simulink model "mod_fm"  (R2024b)
settings: Solver=FixedStepDiscrete  StartTime=0.0  StopTime=0.05  FixedStep=5e-06  RelTol=1e-3
model workspace (MAT data in the model file):
  df = 5000
  fc = 10000
  fm = 1000
  fs = 200000
  hpost = [-1.25061059478e-19 -3.24125186585e-05 -6.55214055151e-05 -9.93614444025e-05 -0.000133925361151 -0.000169142005337 -0.000204855936976 -0.00024080932373 -0.0002766270145 -0.000311805588382 -0.000345707084751 -0.000377558002721 ... (201 elements, 1x201)]
  hpre = [-2.4993987069e-19 -6.42670110592e-05 -0.000126833377255 -0.000184633240487 -0.000234548351952 -0.000273478101959 -0.00029844948245 -0.000306771591638 -0.000296232329902 -0.000265327256793 -0.000213503048842 -0.000141391531522 ... (201 elements, 1x201)]
  phi = 0.7
  sigma2 = 0.02
undefined symbols (not defined in the file): DiscIntNeverNeededParam
settings Model: Creator=runner  LastModifiedBy=runner

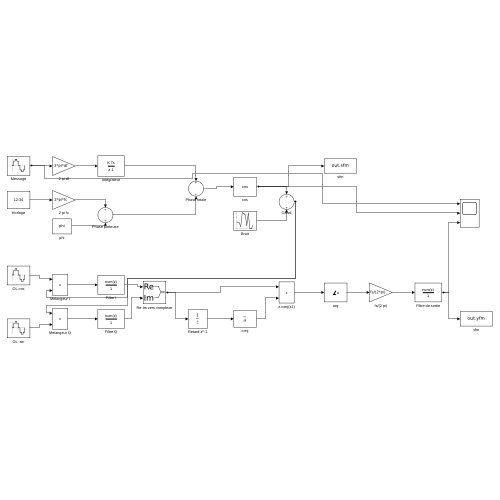
[thumbnail: Simulink's stored preview of the top-level diagram]
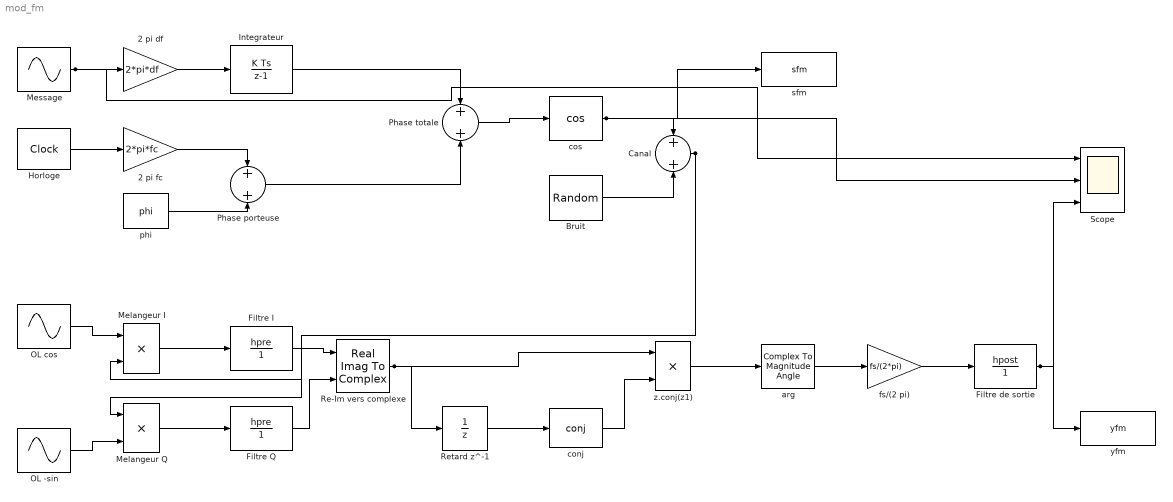
== system mod_fm ==
  2 pi df : Gain  Gain=2*pi*df
  2 pi fc : Gain  Gain=2*pi*fc
  Bruit : RandomNumber  Variance=sigma2  Seed=1  SampleTime=1/fs
  Canal : Sum
  Filtre I : DiscreteFilter  Numerator=hpre  Denominator=1
  Filtre Q : DiscreteFilter  Numerator=hpre  Denominator=1
  Filtre de sortie : DiscreteFilter  Numerator=hpost  Denominator=1
  Horloge : DigitalClock  SampleTime=1/fs
  Integrateur : DiscreteIntegrator  gainval=1  SampleTime=1/fs  ICPrevOutput=DiscIntNeverNeededParam  ICPrevScaledInput=DiscIntNeverNeededParam
  Melangeur I : Product
  Melangeur Q : Product
  Message : Sin  Frequency=2*pi*fm  Phase=pi/2  SampleTime=1/fs
  OL -sin : Sin  Amplitude=-2  Frequency=2*pi*fc  SampleTime=1/fs
  OL cos : Sin  Amplitude=2  Frequency=2*pi*fc  Phase=pi/2  SampleTime=1/fs
  Phase porteuse : Sum
  Phase totale : Sum
  Re-Im vers complexe : RealImagToComplex
  Retard z^-1 : UnitDelay  SampleTime=-1  HasFrameUpgradeWarning=on
  Scope : Scope  NumInputPorts=3
  arg : ComplexToMagnitudeAngle  Output=Angle
  conj : Math  Operator=conj
  cos : Trigonometry  Operator=cos
  fs/(2 pi) : Gain  Gain=fs/(2*pi)
  phi : Constant  Value=phi
  sfm : ToWorkspace  VariableName=sfm  SampleTime=-1
  yfm : ToWorkspace  VariableName=yfm  SampleTime=-1
  z.conj(z1) : Product
  wires:
  Message/1 -> 2 pi df/1, Scope/1
  2 pi df/1 -> Integrateur/1
  Horloge/1 -> 2 pi fc/1
  2 pi fc/1 -> Phase porteuse/1
  phi/1 -> Phase porteuse/2
  Integrateur/1 -> Phase totale/1
  Phase porteuse/1 -> Phase totale/2
  Phase totale/1 -> cos/1
  cos/1 -> Canal/1, sfm/1, Scope/2
  Bruit/1 -> Canal/2
  OL cos/1 -> Melangeur I/1
  Canal/1 -> Melangeur I/2, Melangeur Q/1
  OL -sin/1 -> Melangeur Q/2
  Melangeur I/1 -> Filtre I/1
  Melangeur Q/1 -> Filtre Q/1
  Filtre I/1 -> Re-Im vers complexe/1
  Filtre Q/1 -> Re-Im vers complexe/2
  Re-Im vers complexe/1 -> Retard z^-1/1, z.conj(z1)/1
  Retard z^-1/1 -> conj/1
  conj/1 -> z.conj(z1)/2
  z.conj(z1)/1 -> arg/1
  arg/1 -> fs/(2 pi)/1
  fs/(2 pi)/1 -> Filtre de sortie/1
  Filtre de sortie/1 -> yfm/1, Scope/3
